simulink model "DCHR_Capacity_Chain_Stateflow_v63"  (R2026a)
settings: Solver=FixedStepDiscrete  StopTime=6  FixedStep=1
model workspace (MAT data in the model file):
  charge_cfg_v63 = [0  3  1  0.9  0  0.2  20  45  2  2  5  35  5  5  0.5  0.5  30  20  40  70  0.1  0.2  0.21  8.22777777878  63  2.20703125  2.2265625  1  0  1  0  0  7.77777777678  7.77777777878  0.25; 1  3  1  0.9  0  0.2  20  45  2  2  5  35  5  5  0.5  0.5  30  20  40  70  0.1  0.2  0.21  8.22777777878  63  2.20703125  2.2265625  1  0  1  0  0  7.77777777678  7.77777777878  0.25; 2  3  1  0.9  0  0.2  20  45  2  2  5  35  5  5  0.5  0.5  30  20  40  70  0.1  0.2  0.21  8.22777777878  63  2.20703125  2.2265625  1  0  1  0  0  7.77777777678  7.77777777878  0.25; 3  3  1  0.9  0  0.2  20  45  2  2  5  35  5  5  0.5  0.5  30  20  40  70  0.1  0.2  0.21  8.22777777878  63  2.20703125  2.2265625  1  0  1  0  0  7.77777777678  7.77777777878  0.25; 4  3  1  0.9  0  0.2  20  45  2  2  5  35  5  5  0.5  0.5  30  20  40  70  0.1  0.2  0.21  8.22777777878  63  2.20703125  2.2265625  1  0  1  0  0  7.77777777678  7.77777777878  0.25; 5  3  1  0.9  0  0.2  20  45  2  2  5  35  5  5  0.5  0.5  30  20  40  70  0.1  0.2  0.21  8.22777777878  63  2.20703125  2.2265625  1  0  1  0  0  7.77777777678  7.77777777878  0.25; 6  3  1  0.9  0  0.2  20  45  2  2  5  35  5  5  0.5  0.5  30  20  40  70  0.1  0.2  0.21  8.22777777878  63  2.20703125  2.2265625  1  0  1  0  0  7.77777777678  7.77777777878  0.25]
  charge_steps_v63 = [0  0  0  0; 1  1  0  0; 2  2  5.00217013839  0; 3  3  0  0; 4  4  7.90277777878  0; 5  4  8.02777777778  0; 6  4  8.22777777878  0]
settings Model: Creator=Lysda  LastModifiedBy=Lysda

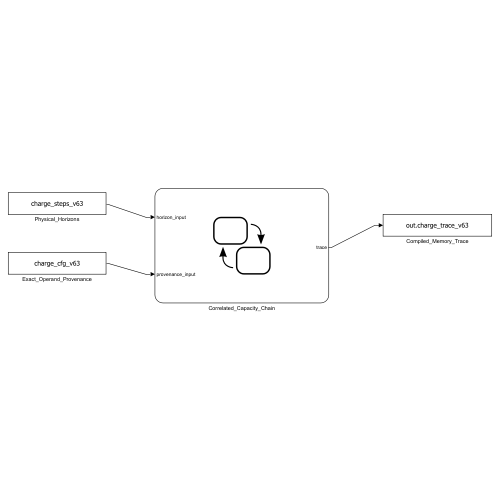
[thumbnail: Simulink's stored preview of the top-level diagram]
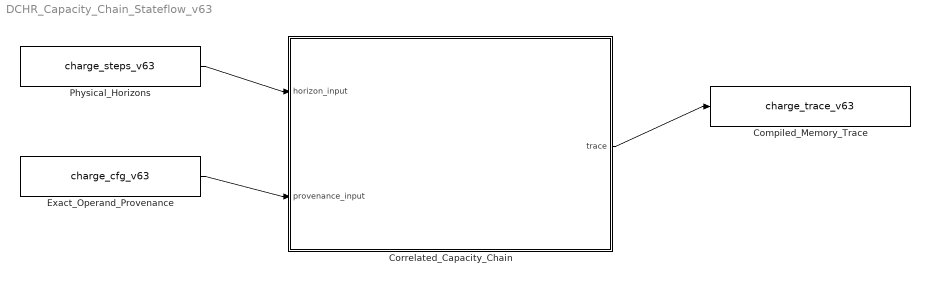
== system DCHR_Capacity_Chain_Stateflow_v63 ==
  Compiled_Memory_Trace : ToWorkspace  VariableName=charge_trace_v63  SaveFormat=Timeseries  SampleTime=-1
  Correlated_Capacity_Chain : Stateflow chart  TreatAsAtomicUnit=on
  Exact_Operand_Provenance : FromWorkspace  VariableName=charge_cfg_v63  SampleTime=1  Interpolate=off  OutputAfterFinalValue=Holding final value
  Physical_Horizons : FromWorkspace  VariableName=charge_steps_v63  SampleTime=1  Interpolate=off  OutputAfterFinalValue=Holding final value
  wires:
  Physical_Horizons/1 -> Correlated_Capacity_Chain/1(horizon_input)
  Exact_Operand_Provenance/1 -> Correlated_Capacity_Chain/2(provenance_input)
  Correlated_Capacity_Chain/1(trace) -> Compiled_Memory_Trace/1

== stateflow chart DCHR_Capacity_Chain_Stateflow_v63/Correlated_Capacity_Chain ==
  settings: description=v63 fixed 80-double correlated capacity chain; compiled global flow and tank-linked source/water ports. Five protocol phases, not solver-clock physical event firing. Exact operand expression retained, enclosures only, constant request upward branch.
  state FLOOR_CHARGE
    en:
    trace=charge_memory_kernel_v63(horizon_input,provenance_input,retained_memory,0);
    retained_memory=trace;
    du:
    trace=charge_memory_kernel_v63(horizon_input,provenance_input,retained_memory,0);
    retained_memory=trace;
  state CORRELATED_CONTACT
    en:
    trace=charge_memory_kernel_v63(horizon_input,provenance_input,retained_memory,1);
    retained_memory=trace;
    du:
    trace=charge_memory_kernel_v63(horizon_input,provenance_input,retained_memory,1);
    retained_memory=trace;
  state TANK_CHARGE
    en:
    trace=charge_memory_kernel_v63(horizon_input,provenance_input,retained_memory,2);
    retained_memory=trace;
    du:
    trace=charge_memory_kernel_v63(horizon_input,provenance_input,retained_memory,2);
    retained_memory=trace;
  state CAPACITY_CONTACT
    en:
    trace=charge_memory_kernel_v63(horizon_input,provenance_input,retained_memory,3);
    retained_memory=trace;
    du:
    trace=charge_memory_kernel_v63(horizon_input,provenance_input,retained_memory,3);
    retained_memory=trace;
  state PASSIVE_COOLING
    en:
    trace=charge_memory_kernel_v63(horizon_input,provenance_input,retained_memory,4);
    retained_memory=trace;
    du:
    trace=charge_memory_kernel_v63(horizon_input,provenance_input,retained_memory,4);
    retained_memory=trace;
  (default) -> FLOOR_CHARGE
  FLOOR_CHARGE -> CORRELATED_CONTACT : [horizon_input(1)==1]
  CORRELATED_CONTACT -> TANK_CHARGE : [horizon_input(1)==2]
  TANK_CHARGE -> CAPACITY_CONTACT : [horizon_input(1)==3]
  CAPACITY_CONTACT -> PASSIVE_COOLING : [horizon_input(1)==4]
  data: step function_input; cfg function_input; previous function_input; stage function_input; y function_output; horizon_input input double size=[3 1]; provenance_input input double size=[34 1]; trace output double size=[80 1]; retained_memory local double size=[80 1] =zeros(80,1)
  function y=charge_memory_kernel_v63(step,cfg,previous,stage):
    | function y=charge_memory_kernel_v63(step,cfg,previous,stage)
    | %#codegen
    | % Fixed-size compiled correlated charge memory. See v63 schema/derivation.
    | % Original binary operands define the exact manifold; no scalar event reset.
    | assert(all(isfinite(cfg))&&all(isfinite(step)),'v63 finite input required');
    | assert(step(1)==stage,'v63 phase mismatch');
    | assert(numel(cfg)==34&&cfg(34)>0,'v63 OFF dwell domain');
    | assert(step(3)==0,'v63 restart unsupported: OFF dwell and restart integration required');
    | assert(cfg(2)>0&&cfg(3)>0&&cfg(3)<=1&&cfg(4)>=0&&cfg(5)>0,'v63 ODE domain');
    | assert(cfg(13)>0&&cfg(14)>0&&cfg(15)>0&&cfg(16)>0&&cfg(17)>0&&cfg(18)>0,'v63 equipment domain');
    | assert(cfg(20)>=0&&cfg(21)>=0&&cfg(21)<=cfg(22),'v63 auxiliary/age domain');
    | assert(cfg(25)>0&&cfg(25)<cfg(26)&&cfg(26)<cfg(23),'v63 event time domain');
    | assert(all(cfg(27:31)==0|cfg(27:31)==1)&&cfg(27)==1&&cfg(30)==0,'v63 tie domain');
    | assert(cfg(24)==63,'v63 schema version');
    | if stage>0
    |     assert(all(cfg(1:31)==previous(1:31))&&all(cfg(32:34)==previous(65:67)),'v63 immutable manifold provenance');
    |     assert(previous(56)==0&&previous(57)==63,'v63 memory authorization');
    | end
    | P=@(v)[v v];
    | C=P(cfg(5));Ta=P(cfg(6));F=plusiv(P(cfg(7)),P(cfg(8)));d=P(cfg(9));
    | star=muliv(C,minusiv(minusiv(F,Ta),d));cap=muliv(C,minusiv(P(cfg(19)),Ta));
    | Te=minusiv(minusiv(P(cfg(11)),P(cfg(12))),P(cfg(13)));
    | a=muliv(P(cfg(14)),plusiv(Te,P(273.15)));
    | lf=minusiv(plusiv(F,P(cfg(10))),Te);
    | l0=minusiv(plusiv(plusiv(Ta,d),P(cfg(10))),Te);
    | assert(a(1)>0&&lf(1)>0&&star(1)>cfg(1)&&cap(1)>star(2),'v63 thermal domain');
    | B=muliv(P(cfg(3)),P(cfg(2)));k=-P(cfg(4));
    | assert(minusiv(B,muliv(P(cfg(4)),cap))*[1;0]>0,'v63 increasing whole trajectory required');
    | % Certify incoming/outgoing sides using the compiled flow, not host port data.
    | [elo,~]=flow(P(cfg(1)),P(cfg(25)),k,B);
    | [ehi,~]=flow(P(cfg(1)),P(cfg(26)),k,B);
    | assert(elo(2)<star(1)&&ehi(1)>star(2),'v63 event bracket not certified');
    | % The host exact-rational adapter certifies equivalent ties; compiled checks
    | % strict non-ties and interval equality consistency, never chooses a tie by eps.
    | limits=zeros(5,2);limits(1,:)=P(cfg(2));limits(2,:)=P(cfg(16));
    | limits(3,:)=muliv(P(cfg(15)),d);
    | limits(4,:)=muliv(muliv(P(cfg(17)),P(cfg(12))),plusiv(P(1),diviv(lf,a)));
    | limits(5,:)=P(cfg(18));
    | for j=1:5
    |     if cfg(26+j)==1
    |         assert(limits(j,1)<=cfg(2)&&limits(j,2)>=cfg(2),'v63 inconsistent equivalent tie');
    |     else
    |         assert(limits(j,1)>cfg(2),'v63 strict request limiter unresolved');
    |     end
    | end
    | [clo,~]=flow(P(cfg(1)),P(cfg(32)),k,B);
    | [chi,~]=flow(P(cfg(1)),P(cfg(33)),k,B);
    | assert(cfg(26)<cfg(32)&&cfg(32)<cfg(33)&&cfg(33)<cfg(23),'v63 capacity event ordering');
    | assert(clo(2)<cap(1)&&chi(1)>cap(2),'v63 capacity bracket not certified');
    | if stage==0
    |     assert(step(2)==0&&previous(57)==0,'v63 initial memory required');t=P(0);
    | elseif stage==1
    |     assert(previous(34)==0&&step(2)==0,'v63 contact sequence');t=cfg(25:26)';
    | elseif stage==2
    |     assert(stage==2&&(previous(34)==1||previous(34)==2),'v63 outgoing sequence');
    |     assert(step(2)>cfg(26)&&step(2)>previous(36)&&step(2)<=cfg(23),'v63 physical horizon must advance');
    |     t=P(step(2));
    |     assert(t(2)<cfg(32),'v63 active horizon crosses capacity event');
    | elseif stage==3
    |     assert(previous(34)==2&&step(2)==0,'v63 capacity contact sequence');
    |     t=cfg(32:33)';
    | else
    |     assert(stage==4&&(previous(34)==3||previous(34)==4),'v63 passive sequence');
    |     assert(step(2)>cfg(33)&&step(2)>previous(36)&&step(2)<=cfg(23),'v63 passive physical horizon must advance');
    |     t=cfg(32:33)';
    | end
    | [en,integral]=flow(P(cfg(1)),t,k,B);
    | if stage==1
    |     % Contact has the symbolic exact star, while root enclosure is retained.
    |     en=star;
    | elseif stage==2
    |     assert(en(1)>star(2),'v63 outgoing branch unresolved');
    | end
    | if stage>=3,en=cap;end
    | assert(en(1)>=0&&(stage>=3||en(2)<cap(1)),'v63 TES bounds');
    | heat=muliv(P(cfg(2)),t);source=P(0);
    | % Global-time rectangles include the uncertain event window. The continuous
    | % max(floor,Ttank+approach) water law avoids a scalar branch handoff.
    | for j=1:128
    |     t0=muliv(t,diviv(P(j-1),P(128)));t1=muliv(t,diviv(P(j),P(128)));
    |     [e0,~]=flow(P(cfg(1)),t0,k,B);[e1,~]=flow(P(cfg(1)),t1,k,B);
    |     ecell=[e0(1) e1(2)];lift=plusiv(l0,diviv(ecell,C));lift=[max(lf(1),lift(1)) max(lf(2),lift(2))];
    |     rate=muliv(P(cfg(2)),diviv(a,plusiv(a,lift)));
    |     source=plusiv(source,muliv(rate,diviv(t,P(128))));
    | end
    | work=minusiv(heat,source);standing=muliv(P(cfg(4)),integral);
    | chargeLoss=muliv(minusiv(P(1),P(cfg(3))),heat);aux=muliv(P(cfg(20)),work);
    | offage=P(0);ready=0;latch=1;
    | if stage>=3,latch=0;end
    | if stage==4
    |     offage=minusiv(P(step(2)),cfg(32:33)');
    |     assert(offage(1)>0,'v63 OFF clock unresolved');
    |     [en,~]=flow(cap,offage,k,P(0));
    |     if cfg(4)>0,standing=plusiv(standing,minusiv(cap,en));end
    |     if cfg(4)==0,en=cap;end
    |     assert(en(1)>=0&&en(2)<=cap(2),'v63 passive TES bounds');
    |     if offage(1)>=cfg(34),ready=1;elseif offage(2)>=cfg(34),ready=2;end
    | end
    | law=minusiv(minusiv(minusiv(plusiv(P(cfg(1)),heat),en),standing),chargeLoss);
    | assert(source(1)>=0&&work(1)>=0&&standing(1)>=0&&chargeLoss(1)>=0,'v63 nonnegative ports');
    | assert(law(1)<=0&&law(2)>=0,'v63 first law enclosure');
    | age=plusiv(cfg(21:22)',t);
    | if stage>0,assert(age(1)>=previous(39)&&age(2)>=previous(40),'v63 HP clock reset');end
    | if stage==4,t=P(step(2));end
    | temp=plusiv(Ta,diviv(en,C));hot=[max(F(1),temp(1)+cfg(9)) max(F(2),temp(2)+cfg(9))];
    | if stage>0,waterFlow=diviv(P(cfg(2)),d);else,waterFlow=diviv(P(cfg(2)),minusiv(F,temp));end
    | if stage>=3
    |     waterFlow=P(0);hot=P(0);
    | elseif cfg(29)==1&&stage>0
    |     % Exact host certificate q=H*d; same d expression, no subtractive decorrelation.
    |     assert(waterFlow(1)<=cfg(15)&&waterFlow(2)>=cfg(15),'v63 finite hot-water tie');
    | else
    |     assert(waterFlow(1)>=0&&waterFlow(2)<=cfg(15),'v63 finite hot-water capacity');
    | end
    | if stage>=3,waterFlow=P(0);hot=P(0);end
    | y=zeros(80,1);y(1:31)=cfg(1:31);y(32:33)=star';y(34)=stage;y(35:36)=t';
    | y(37:38)=en';y(39:40)=age';y(41:42)=heat';y(43:44)=source';y(45:46)=work';
    | y(47:48)=standing';y(49:50)=chargeLoss';y(51:52)=aux';y(53:54)=law';
    | y(55)=latch;y(56)=0;y(57)=63;y(58:59)=cap';y(60:61)=waterFlow';y(62:63)=hot';y(64)=128;y(65:67)=cfg(32:34);y(68:69)=cfg(32:33);y(70:71)=offage';y(72)=ready;
    | y(73)=3;y(74:75)=cfg(21:22);y(76:77)=cfg(25:26);y(78:79)=cap';y(80)=0;
    | end
    | function [en,integral]=flow(initial,t,k,B)
    | if all(t==0),en=initial;integral=[0 0];return;end
    | x=muliv(k,t);assert(max(abs(x))<=1,'v63 outward span exceeds one');
    | v=plusiv(muliv(k,initial),B);f1=[1 1];f2=[.5 .5];term=[1 1];
    | for ii=1:24,term=diviv(muliv(term,x),[ii+1 ii+1]);f1=plusiv(f1,term);f2=plusiv(f2,diviv(term,[ii+2 ii+2]));end
    | fac=[1 1];for ii=2:26,fac=muliv(fac,[ii ii]);end
    | tail=diviv([3 3],fac);f1=plusiv(f1,[-tail(2) tail(2)]);f2=plusiv(f2,[-tail(2) tail(2)]);
    | en=plusiv(initial,muliv(muliv(v,t),f1));integral=plusiv(muliv(initial,t),muliv(muliv(v,muliv(t,t)),f2));
    | end
    | function z=plusiv(x,y)
    | if all(x==0),z=y;elseif all(y==0),z=x;else,z=out([x(1)+y(1) x(2)+y(2)]);end
    | end
    | function z=minusiv(x,y)
    | if all(y==0),z=x;elseif x(1)==x(2)&&y(1)==y(2)&&x(1)==y(1),z=[0 0];else,z=out([x(1)-y(2) x(2)-y(1)]);end
    | end
    | function z=muliv(x,y)
    | if all(x==0)||all(y==0),z=[0 0];return;end
    | t=[x(1)*y(1) x(1)*y(2) x(2)*y(1) x(2)*y(2)];z=out([min(t) max(t)]);
    | end
    | function z=diviv(x,y)
    | assert(y(1)>0,'v63 positive denominator required');
    | if all(x==0),z=[0 0];return;end
    | t=[x(1)/y(1) x(1)/y(2) x(2)/y(1) x(2)/y(2)];z=out([min(t) max(t)]);
    | end
    | function z=out(t)
    | assert(all(isfinite(t)),'v63 arithmetic overflow');z=[t(1)-2*eps(t(1)) t(2)+2*eps(t(2))];
    | assert(all(isfinite(z))&&z(1)<=z(2),'v63 expansion overflow');
    | end
